simulink model "sm_abbYuMi_trajectory"  (R2025a)
settings: Solver=daessc  StartTime=0.0  StopTime=size(waypointsL,2)*segment_duration  MaxStep=0.5  RelTol=1e-3  AbsTol=1e-3
values from neighbouring files (symbols this model uses):
  cube_l = 0.02    [startup_sm_abbYuMi_trajectory.m]
  segment_duration = 2    [startup_sm_abbYuMi_trajectory.m]
undefined symbols (not defined in the file or in its folder): F1, F2, X, Y, Z
libraries: sm_lib x210, nesl_utility x31, robotcorelib x2
(part 2 of 5)

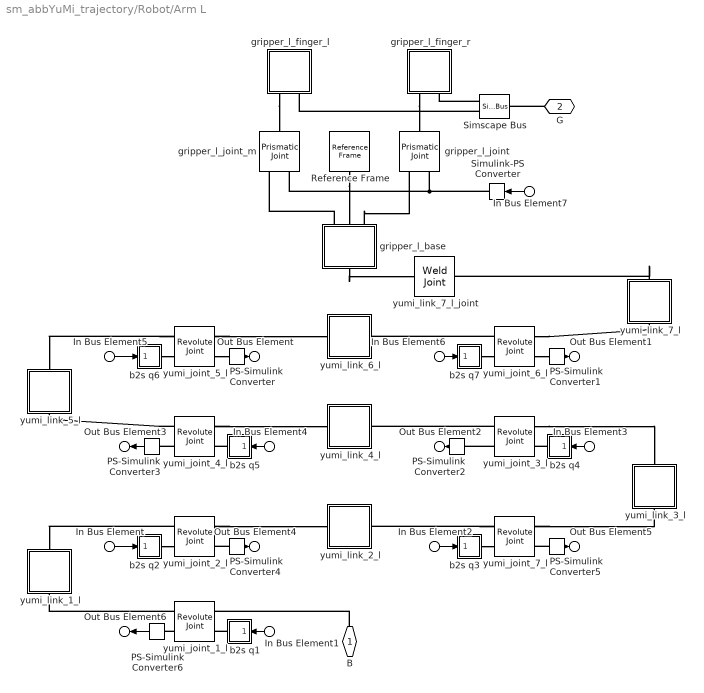
== system sm_abbYuMi_trajectory/Robot/Arm L ==
  In Bus Element1 : Inport  PortName=q  Element=q1
  In Bus Element : Inport  PortName=q  Element=q2
  In Bus Element2 : Inport  PortName=q  Element=q3
  In Bus Element3 : Inport  PortName=q  Element=q4
  In Bus Element4 : Inport  PortName=q  Element=q5
  In Bus Element5 : Inport  PortName=q  Element=q6
  In Bus Element6 : Inport  PortName=q  Element=q7
  In Bus Element7 : Inport  PortName=q  Element=f
  PS-Simulink Converter{,1..6} (7 alike) : nesl_utility/PS-Simulink Converter  PhysicalDomain=network_engine_domain  SubClassName=ps_output  LeftPortType=input  RightPortType=output  PseudoPeriodic=off  Frequencies=[]  VectorFormat=1-D array  Unit=inherit  AffineConversion=off
  Reference Frame : sm_lib/Frames and Transforms/Reference Frame
  Simscape Bus : SimscapeBus  HierarchyStrings=F1;F2
  Simulink-PS Converter : nesl_utility/Simulink-PS Converter  PhysicalDomain=network_engine_domain  SubClassName=ps_input  LeftPortType=input  RightPortType=output  PseudoPeriodic=off  Frequencies=[]  NoiseDistribution=none  NoiseParameters=[]  Unit=m  AffineConversion=off  FilteringAndDerivatives=filter  SimscapeFilterOrder=2  InputFilterTimeConstant=0.1  UdotUserProvided=0
  b2s q1 : Subsystem
  b2s q2 : Subsystem
  b2s q3 : Subsystem
  b2s q4 : Subsystem
  b2s q5 : Subsystem
  b2s q6 : Subsystem
  b2s q7 : Subsystem
  gripper_l_base : Subsystem
  gripper_l_finger_l : Subsystem
  gripper_l_finger_r : Subsystem
  gripper_l_joint : sm_lib/Joints/Prismatic Joint  JointMode=Normal  CompositeWrenchDir=FollowerOnBase  CompositeWrenchFrame=BaseFrame  SenseConstraintForce=off  SenseConstraintTorque=off  SenseTotalForce=off  SenseTotalTorque=off  PositionTargetSpecify=off  PositionTargetPriority=High  PositionTargetValue=0  PositionTargetValueUnits=m  VelocityTargetSpecify=off  VelocityTargetPriority=High  VelocityTargetValue=0  VelocityTargetValueUnits=m/s  EquilibriumPosition=0  EquilibriumPositionUnits=m  SpringStiffness=0  SpringStiffnessUnits=N/m  DampingCoefficient=1  DampingCoefficientUnits=kg/s  LowerLimitSpecify=on  LowerLimitBound=0  LowerLimitBoundUnits=m  LowerLimitStiffness=1e6  LowerLimitStiffnessUnits=N/m  LowerLimitDamping=1e3  LowerLimitDampingUnits=N/(m/s)  LowerLimitTransitionRegionWidth=1e-4  LowerLimitTransitionRegionWidthUnits=m  UpperLimitSpecify=on  UpperLimitBound=0.025  UpperLimitBoundUnits=m  UpperLimitStiffness=1e6  UpperLimitStiffnessUnits=N/m  UpperLimitDamping=1e3  UpperLimitDampingUnits=N/(m/s)  UpperLimitTransitionRegionWidth=1e-4  UpperLimitTransitionRegionWidthUnits=m  TorqueActuationMode=ComputedTorque  MotionActuationMode=InputMotion  SensePosition=off  SenseVelocity=off  SenseAcceleration=off  SenseTorqueForce=off  SenseLowerLimitTorqueForce=off  SenseUpperLimitTorqueForce=off
  gripper_l_joint_m : sm_lib/Joints/Prismatic Joint  JointMode=Normal  CompositeWrenchDir=FollowerOnBase  CompositeWrenchFrame=BaseFrame  SenseConstraintForce=off  SenseConstraintTorque=off  SenseTotalForce=off  SenseTotalTorque=off  PositionTargetSpecify=off  PositionTargetPriority=High  PositionTargetValue=0  PositionTargetValueUnits=m  VelocityTargetSpecify=off  VelocityTargetPriority=High  VelocityTargetValue=0  VelocityTargetValueUnits=m/s  EquilibriumPosition=0  EquilibriumPositionUnits=m  SpringStiffness=0  SpringStiffnessUnits=N/m  DampingCoefficient=1  DampingCoefficientUnits=kg/s  LowerLimitSpecify=on  LowerLimitBound=0  LowerLimitBoundUnits=m  LowerLimitStiffness=1e6  LowerLimitStiffnessUnits=N/m  LowerLimitDamping=1e3  LowerLimitDampingUnits=N/(m/s)  LowerLimitTransitionRegionWidth=1e-4  LowerLimitTransitionRegionWidthUnits=m  UpperLimitSpecify=on  UpperLimitBound=0.025  UpperLimitBoundUnits=m  UpperLimitStiffness=1e6  UpperLimitStiffnessUnits=N/m  UpperLimitDamping=1e3  UpperLimitDampingUnits=N/(m/s)  UpperLimitTransitionRegionWidth=1e-4  UpperLimitTransitionRegionWidthUnits=m  TorqueActuationMode=ComputedTorque  MotionActuationMode=InputMotion  SensePosition=off  SenseVelocity=off  SenseAcceleration=off  SenseTorqueForce=off  SenseLowerLimitTorqueForce=off  SenseUpperLimitTorqueForce=off
  yumi_joint_1_l : sm_lib/Joints/Revolute Joint  JointMode=Normal  CompositeWrenchDir=FollowerOnBase  CompositeWrenchFrame=BaseFrame  SenseConstraintForce=off  SenseConstraintTorque=off  SenseTotalForce=off  SenseTotalTorque=off  PositionTargetSpecify=on  PositionTargetPriority=High  PositionTargetValue=45  PositionTargetValueUnits=deg  VelocityTargetSpecify=off  VelocityTargetPriority=High  VelocityTargetValue=0  VelocityTargetValueUnits=deg/s  EquilibriumPosition=0  EquilibriumPositionUnits=deg  SpringStiffness=0  SpringStiffnessUnits=N*m/deg  DampingCoefficient=0.5  DampingCoefficientUnits=m^2*kg/s/rad  LowerLimitSpecify=on  LowerLimitBound=-2.94087978961  LowerLimitBoundUnits=rad  LowerLimitStiffness=1e4  LowerLimitStiffnessUnits=N*m/deg  LowerLimitDamping=10  LowerLimitDampingUnits=N*m/(deg/s)  LowerLimitTransitionRegionWidth=0.1  LowerLimitTransitionRegionWidthUnits=deg  UpperLimitSpecify=on  UpperLimitBound=2.94087978961  UpperLimitBoundUnits=rad  UpperLimitStiffness=1e4  UpperLimitStiffnessUnits=N*m/deg  UpperLimitDamping=10  UpperLimitDampingUnits=N*m/(deg/s)  UpperLimitTransitionRegionWidth=0.1  UpperLimitTransitionRegionWidthUnits=deg  TorqueActuationMode=ComputedTorque  MotionActuationMode=InputMotion  SensePosition=off  SenseVelocity=off  SenseAcceleration=off  SenseTorqueForce=on  SenseLowerLimitTorqueForce=off  SenseUpperLimitTorqueForce=off
  yumi_joint_2_l : sm_lib/Joints/Revolute Joint  JointMode=Normal  CompositeWrenchDir=FollowerOnBase  CompositeWrenchFrame=BaseFrame  SenseConstraintForce=off  SenseConstraintTorque=off  SenseTotalForce=off  SenseTotalTorque=off  PositionTargetSpecify=off  PositionTargetPriority=High  PositionTargetValue=0  PositionTargetValueUnits=deg  VelocityTargetSpecify=off  VelocityTargetPriority=High  VelocityTargetValue=0  VelocityTargetValueUnits=deg/s  EquilibriumPosition=0  EquilibriumPositionUnits=deg  SpringStiffness=0  SpringStiffnessUnits=N*m/deg  DampingCoefficient=0.5  DampingCoefficientUnits=m^2*kg/s/rad  LowerLimitSpecify=on  LowerLimitBound=-2.50454747661  LowerLimitBoundUnits=rad  LowerLimitStiffness=1e4  LowerLimitStiffnessUnits=N*m/deg  LowerLimitDamping=10  LowerLimitDampingUnits=N*m/(deg/s)  LowerLimitTransitionRegionWidth=0.1  LowerLimitTransitionRegionWidthUnits=deg  UpperLimitSpecify=on  UpperLimitBound=0.759218224618  UpperLimitBoundUnits=rad  UpperLimitStiffness=1e4  UpperLimitStiffnessUnits=N*m/deg  UpperLimitDamping=10  UpperLimitDampingUnits=N*m/(deg/s)  UpperLimitTransitionRegionWidth=0.1  UpperLimitTransitionRegionWidthUnits=deg  TorqueActuationMode=ComputedTorque  MotionActuationMode=InputMotion  SensePosition=off  SenseVelocity=off  SenseAcceleration=off  SenseTorqueForce=on  SenseLowerLimitTorqueForce=off  SenseUpperLimitTorqueForce=off
  yumi_joint_3_l : sm_lib/Joints/Revolute Joint  JointMode=Normal  CompositeWrenchDir=FollowerOnBase  CompositeWrenchFrame=BaseFrame  SenseConstraintForce=off  SenseConstraintTorque=off  SenseTotalForce=off  SenseTotalTorque=off  PositionTargetSpecify=off  PositionTargetPriority=High  PositionTargetValue=0  PositionTargetValueUnits=deg  VelocityTargetSpecify=off  VelocityTargetPriority=High  VelocityTargetValue=0  VelocityTargetValueUnits=deg/s  EquilibriumPosition=0  EquilibriumPositionUnits=deg  SpringStiffness=0  SpringStiffnessUnits=N*m/deg  DampingCoefficient=0.5  DampingCoefficientUnits=m^2*kg/s/rad  LowerLimitSpecify=on  LowerLimitBound=-2.15548162621  LowerLimitBoundUnits=rad  LowerLimitStiffness=1e4  LowerLimitStiffnessUnits=N*m/deg  LowerLimitDamping=10  LowerLimitDampingUnits=N*m/(deg/s)  LowerLimitTransitionRegionWidth=0.1  LowerLimitTransitionRegionWidthUnits=deg  UpperLimitSpecify=on  UpperLimitBound=1.3962634016  UpperLimitBoundUnits=rad  UpperLimitStiffness=1e4  UpperLimitStiffnessUnits=N*m/deg  UpperLimitDamping=10  UpperLimitDampingUnits=N*m/(deg/s)  UpperLimitTransitionRegionWidth=0.1  UpperLimitTransitionRegionWidthUnits=deg  TorqueActuationMode=ComputedTorque  MotionActuationMode=InputMotion  SensePosition=off  SenseVelocity=off  SenseAcceleration=off  SenseTorqueForce=on  SenseLowerLimitTorqueForce=off  SenseUpperLimitTorqueForce=off
  yumi_joint_4_l : sm_lib/Joints/Revolute Joint  JointMode=Normal  CompositeWrenchDir=FollowerOnBase  CompositeWrenchFrame=BaseFrame  SenseConstraintForce=off  SenseConstraintTorque=off  SenseTotalForce=off  SenseTotalTorque=off  PositionTargetSpecify=off  PositionTargetPriority=High  PositionTargetValue=0  PositionTargetValueUnits=deg  VelocityTargetSpecify=off  VelocityTargetPriority=High  VelocityTargetValue=0  VelocityTargetValueUnits=deg/s  EquilibriumPosition=0  EquilibriumPositionUnits=deg  SpringStiffness=0  SpringStiffnessUnits=N*m/deg  DampingCoefficient=0.5  DampingCoefficientUnits=m^2*kg/s/rad  LowerLimitSpecify=on  LowerLimitBound=-5.06145483078  LowerLimitBoundUnits=rad  LowerLimitStiffness=1e4  LowerLimitStiffnessUnits=N*m/deg  LowerLimitDamping=10  LowerLimitDampingUnits=N*m/(deg/s)  LowerLimitTransitionRegionWidth=0.1  LowerLimitTransitionRegionWidthUnits=deg  UpperLimitSpecify=on  UpperLimitBound=5.06145483078  UpperLimitBoundUnits=rad  UpperLimitStiffness=1e4  UpperLimitStiffnessUnits=N*m/deg  UpperLimitDamping=10  UpperLimitDampingUnits=N*m/(deg/s)  UpperLimitTransitionRegionWidth=0.1  UpperLimitTransitionRegionWidthUnits=deg  TorqueActuationMode=ComputedTorque  MotionActuationMode=InputMotion  SensePosition=off  SenseVelocity=off  SenseAcceleration=off  SenseTorqueForce=on  SenseLowerLimitTorqueForce=off  SenseUpperLimitTorqueForce=off
  yumi_joint_5_l : sm_lib/Joints/Revolute Joint  JointMode=Normal  CompositeWrenchDir=FollowerOnBase  CompositeWrenchFrame=BaseFrame  SenseConstraintForce=off  SenseConstraintTorque=off  SenseTotalForce=off  SenseTotalTorque=off  PositionTargetSpecify=off  PositionTargetPriority=High  PositionTargetValue=0  PositionTargetValueUnits=deg  VelocityTargetSpecify=off  VelocityTargetPriority=High  VelocityTargetValue=0  VelocityTargetValueUnits=deg/s  EquilibriumPosition=0  EquilibriumPositionUnits=deg  SpringStiffness=0  SpringStiffnessUnits=N*m/deg  DampingCoefficient=0.5  DampingCoefficientUnits=m^2*kg/s/rad  LowerLimitSpecify=on  LowerLimitBound=-1.53588974176  LowerLimitBoundUnits=rad  LowerLimitStiffness=1e4  LowerLimitStiffnessUnits=N*m/deg  LowerLimitDamping=10  LowerLimitDampingUnits=N*m/(deg/s)  LowerLimitTransitionRegionWidth=0.1  LowerLimitTransitionRegionWidthUnits=deg  UpperLimitSpecify=on  UpperLimitBound=2.40855436775  UpperLimitBoundUnits=rad  UpperLimitStiffness=1e4  UpperLimitStiffnessUnits=N*m/deg  UpperLimitDamping=10  UpperLimitDampingUnits=N*m/(deg/s)  UpperLimitTransitionRegionWidth=0.1  UpperLimitTransitionRegionWidthUnits=deg  TorqueActuationMode=ComputedTorque  MotionActuationMode=InputMotion  SensePosition=off  SenseVelocity=off  SenseAcceleration=off  SenseTorqueForce=on  SenseLowerLimitTorqueForce=off  SenseUpperLimitTorqueForce=off
  yumi_joint_6_l : sm_lib/Joints/Revolute Joint  JointMode=Normal  CompositeWrenchDir=FollowerOnBase  CompositeWrenchFrame=BaseFrame  SenseConstraintForce=off  SenseConstraintTorque=off  SenseTotalForce=off  SenseTotalTorque=off  PositionTargetSpecify=off  PositionTargetPriority=High  PositionTargetValue=0  PositionTargetValueUnits=deg  VelocityTargetSpecify=off  VelocityTargetPriority=High  VelocityTargetValue=0  VelocityTargetValueUnits=deg/s  EquilibriumPosition=0  EquilibriumPositionUnits=deg  SpringStiffness=0  SpringStiffnessUnits=N*m/deg  DampingCoefficient=0.5  DampingCoefficientUnits=m^2*kg/s/rad  LowerLimitSpecify=on  LowerLimitBound=-3.99680398707  LowerLimitBoundUnits=rad  LowerLimitStiffness=1e4  LowerLimitStiffnessUnits=N*m/deg  LowerLimitDamping=10  LowerLimitDampingUnits=N*m/(deg/s)  LowerLimitTransitionRegionWidth=0.1  LowerLimitTransitionRegionWidthUnits=deg  UpperLimitSpecify=on  UpperLimitBound=3.99680398707  UpperLimitBoundUnits=rad  UpperLimitStiffness=1e4  UpperLimitStiffnessUnits=N*m/deg  UpperLimitDamping=10  UpperLimitDampingUnits=N*m/(deg/s)  UpperLimitTransitionRegionWidth=0.1  UpperLimitTransitionRegionWidthUnits=deg  TorqueActuationMode=ComputedTorque  MotionActuationMode=InputMotion  SensePosition=off  SenseVelocity=off  SenseAcceleration=off  SenseTorqueForce=on  SenseLowerLimitTorqueForce=off  SenseUpperLimitTorqueForce=off
  yumi_joint_7_l : sm_lib/Joints/Revolute Joint  JointMode=Normal  CompositeWrenchDir=FollowerOnBase  CompositeWrenchFrame=BaseFrame  SenseConstraintForce=off  SenseConstraintTorque=off  SenseTotalForce=off  SenseTotalTorque=off  PositionTargetSpecify=off  PositionTargetPriority=High  PositionTargetValue=0  PositionTargetValueUnits=deg  VelocityTargetSpecify=off  VelocityTargetPriority=High  VelocityTargetValue=0  VelocityTargetValueUnits=deg/s  EquilibriumPosition=0  EquilibriumPositionUnits=deg  SpringStiffness=0  SpringStiffnessUnits=N*m/deg  DampingCoefficient=0.5  DampingCoefficientUnits=m^2*kg/s/rad  LowerLimitSpecify=on  LowerLimitBound=-2.94087978961  LowerLimitBoundUnits=rad  LowerLimitStiffness=1e4  LowerLimitStiffnessUnits=N*m/deg  LowerLimitDamping=10  LowerLimitDampingUnits=N*m/(deg/s)  LowerLimitTransitionRegionWidth=0.1  LowerLimitTransitionRegionWidthUnits=deg  UpperLimitSpecify=on  UpperLimitBound=2.94087978961  UpperLimitBoundUnits=rad  UpperLimitStiffness=1e4  UpperLimitStiffnessUnits=N*m/deg  UpperLimitDamping=10  UpperLimitDampingUnits=N*m/(deg/s)  UpperLimitTransitionRegionWidth=0.1  UpperLimitTransitionRegionWidthUnits=deg  TorqueActuationMode=ComputedTorque  MotionActuationMode=InputMotion  SensePosition=off  SenseVelocity=off  SenseAcceleration=off  SenseTorqueForce=on  SenseLowerLimitTorqueForce=off  SenseUpperLimitTorqueForce=off
  yumi_link_1_l : Subsystem
  yumi_link_2_l : Subsystem
  yumi_link_3_l : Subsystem
  yumi_link_4_l : Subsystem
  yumi_link_5_l : Subsystem
  yumi_link_6_l : Subsystem
  yumi_link_7_l : Subsystem
  yumi_link_7_l_joint : sm_lib/Joints/Weld Joint  JointMode=Normal  CompositeWrenchDir=FollowerOnBase  CompositeWrenchFrame=BaseFrame  SenseConstraintForce=off  SenseConstraintTorque=off  SenseTotalForce=off  SenseTotalTorque=off
  B : PMIOPort  Side=Right
  G : PMIOPort  Port=2  Side=Right
  Out Bus Element : Outport  PortName=trq  Element=j6
  Out Bus Element1 : Outport  PortName=trq  Element=j7
  Out Bus Element2 : Outport  PortName=trq  Element=j4
  Out Bus Element3 : Outport  PortName=trq  Element=j5
  Out Bus Element4 : Outport  PortName=trq  Element=j2
  Out Bus Element5 : Outport  PortName=trq  Element=j3
  Out Bus Element6 : Outport  PortName=trq  Element=j1
  wires:
  In Bus Element1/1 -> b2s q1/1(b)
  In Bus Element/1 -> b2s q2/1(b)
  In Bus Element2/1 -> b2s q3/1(b)
  In Bus Element3/1 -> b2s q4/1(b)
  In Bus Element4/1 -> b2s q5/1(b)
  In Bus Element5/1 -> b2s q6/1(b)
  In Bus Element6/1 -> b2s q7/1(b)
  In Bus Element7/1 -> Simulink-PS Converter/1
  PS-Simulink Converter/1 -> Out Bus Element/1
  PS-Simulink Converter1/1 -> Out Bus Element1/1
  PS-Simulink Converter2/1 -> Out Bus Element2/1
  PS-Simulink Converter3/1 -> Out Bus Element3/1
  PS-Simulink Converter4/1 -> Out Bus Element4/1
  PS-Simulink Converter5/1 -> Out Bus Element5/1
  PS-Simulink Converter6/1 -> Out Bus Element6/1
  connections:
  gripper_l_base/LConn1 -- yumi_link_7_l_joint/RConn1
  gripper_l_finger_l/LConn1 -- gripper_l_joint_m/RConn1
  gripper_l_base/RConn3 -- gripper_l_joint/LConn1
  yumi_joint_1_l/RConn1 -- yumi_link_1_l/LConn1
  yumi_joint_2_l/LConn1 -- yumi_link_1_l/RConn1
  yumi_joint_4_l/RConn1 -- yumi_link_5_l/LConn1
  yumi_link_7_l/RConn1 -- yumi_link_7_l_joint/LConn1
  yumi_joint_4_l/LConn1 -- yumi_link_4_l/RConn1
  yumi_joint_7_l/RConn1 -- yumi_link_3_l/LConn1
  yumi_joint_3_l/RConn1 -- yumi_link_4_l/LConn1
  yumi_joint_2_l/RConn1 -- yumi_link_2_l/LConn1
  yumi_joint_5_l/LConn1 -- yumi_link_5_l/RConn1
  yumi_joint_6_l/LConn1 -- yumi_link_6_l/RConn1
  yumi_joint_5_l/RConn1 -- yumi_link_6_l/LConn1
  gripper_l_base/RConn1 -- gripper_l_joint_m/LConn1
  yumi_joint_3_l/LConn1 -- yumi_link_3_l/RConn1
  gripper_l_finger_r/LConn1 -- gripper_l_joint/RConn1
  yumi_joint_7_l/LConn1 -- yumi_link_2_l/RConn1
  yumi_joint_6_l/RConn1 -- yumi_link_7_l/LConn1
  B/RConn1 -- yumi_joint_1_l/LConn1
  b2s q1/RConn1 -- yumi_joint_1_l/LConn2
  b2s q2/RConn1 -- yumi_joint_2_l/LConn2
  b2s q3/RConn1 -- yumi_joint_7_l/LConn2
  b2s q4/RConn1 -- yumi_joint_3_l/LConn2
  b2s q5/RConn1 -- yumi_joint_4_l/LConn2
  b2s q6/RConn1 -- yumi_joint_5_l/LConn2
  b2s q7/RConn1 -- yumi_joint_6_l/LConn2
  Simulink-PS Converter/RConn1 -- gripper_l_joint/LConn2 -- gripper_l_joint_m/LConn2
  Reference Frame/RConn1 -- gripper_l_base/RConn2
  G/RConn1 -- Simscape Bus/RConn1
  Simscape Bus/LConn1 -- gripper_l_finger_r/LConn2
  Simscape Bus/LConn2 -- gripper_l_finger_l/LConn2
  yumi_joint_5_l/RConn2 -- PS-Simulink Converter/LConn1
  yumi_joint_6_l/RConn2 -- PS-Simulink Converter1/LConn1
  yumi_joint_3_l/RConn2 -- PS-Simulink Converter2/LConn1
  yumi_joint_4_l/RConn2 -- PS-Simulink Converter3/LConn1
  PS-Simulink Converter4/LConn1 -- yumi_joint_2_l/RConn2
  PS-Simulink Converter5/LConn1 -- yumi_joint_7_l/RConn2
  yumi_joint_1_l/RConn2 -- PS-Simulink Converter6/LConn1

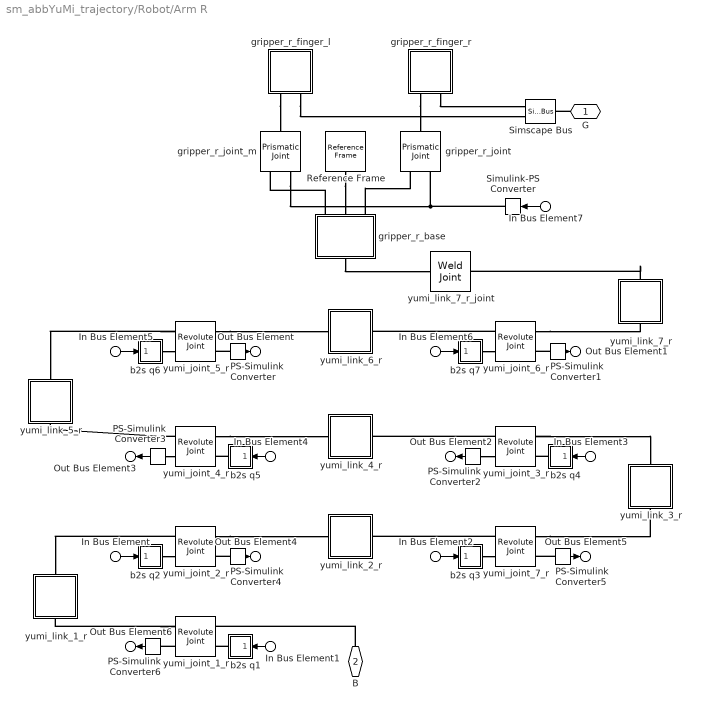
== system sm_abbYuMi_trajectory/Robot/Arm R ==
  In Bus Element1 : Inport  PortName=q  Element=q1
  In Bus Element : Inport  PortName=q  Element=q2
  In Bus Element2 : Inport  PortName=q  Element=q3
  In Bus Element3 : Inport  PortName=q  Element=q4
  In Bus Element4 : Inport  PortName=q  Element=q5
  In Bus Element5 : Inport  PortName=q  Element=q6
  In Bus Element6 : Inport  PortName=q  Element=q7
  In Bus Element7 : Inport  PortName=q  Element=f
  PS-Simulink Converter{,1..6} (7 alike) : nesl_utility/PS-Simulink Converter  PhysicalDomain=network_engine_domain  SubClassName=ps_output  LeftPortType=input  RightPortType=output  PseudoPeriodic=off  Frequencies=[]  VectorFormat=1-D array  Unit=inherit  AffineConversion=off
  Reference Frame : sm_lib/Frames and Transforms/Reference Frame
  Simscape Bus : SimscapeBus  HierarchyStrings=F1;F2
  Simulink-PS Converter : nesl_utility/Simulink-PS Converter  PhysicalDomain=network_engine_domain  SubClassName=ps_input  LeftPortType=input  RightPortType=output  PseudoPeriodic=off  Frequencies=[]  NoiseDistribution=none  NoiseParameters=[]  Unit=m  AffineConversion=off  FilteringAndDerivatives=filter  SimscapeFilterOrder=2  InputFilterTimeConstant=0.1  UdotUserProvided=0
  b2s q1 : Subsystem
  b2s q2 : Subsystem
  b2s q3 : Subsystem
  b2s q4 : Subsystem
  b2s q5 : Subsystem
  b2s q6 : Subsystem
  b2s q7 : Subsystem
  gripper_r_base : Subsystem
  gripper_r_finger_l : Subsystem
  gripper_r_finger_r : Subsystem
  gripper_r_joint : sm_lib/Joints/Prismatic Joint  JointMode=Normal  CompositeWrenchDir=FollowerOnBase  CompositeWrenchFrame=BaseFrame  SenseConstraintForce=off  SenseConstraintTorque=off  SenseTotalForce=off  SenseTotalTorque=off  PositionTargetSpecify=off  PositionTargetPriority=High  PositionTargetValue=0  PositionTargetValueUnits=m  VelocityTargetSpecify=off  VelocityTargetPriority=High  VelocityTargetValue=0  VelocityTargetValueUnits=m/s  EquilibriumPosition=0  EquilibriumPositionUnits=m  SpringStiffness=0  SpringStiffnessUnits=N/m  DampingCoefficient=1  DampingCoefficientUnits=kg/s  LowerLimitSpecify=on  LowerLimitBound=0  LowerLimitBoundUnits=m  LowerLimitStiffness=1e6  LowerLimitStiffnessUnits=N/m  LowerLimitDamping=1e3  LowerLimitDampingUnits=N/(m/s)  LowerLimitTransitionRegionWidth=1e-4  LowerLimitTransitionRegionWidthUnits=m  UpperLimitSpecify=on  UpperLimitBound=0.025  UpperLimitBoundUnits=m  UpperLimitStiffness=1e6  UpperLimitStiffnessUnits=N/m  UpperLimitDamping=1e3  UpperLimitDampingUnits=N/(m/s)  UpperLimitTransitionRegionWidth=1e-4  UpperLimitTransitionRegionWidthUnits=m  TorqueActuationMode=ComputedTorque  MotionActuationMode=InputMotion  SensePosition=off  SenseVelocity=off  SenseAcceleration=off  SenseTorqueForce=off  SenseLowerLimitTorqueForce=off  SenseUpperLimitTorqueForce=off
  gripper_r_joint_m : sm_lib/Joints/Prismatic Joint  JointMode=Normal  CompositeWrenchDir=FollowerOnBase  CompositeWrenchFrame=BaseFrame  SenseConstraintForce=off  SenseConstraintTorque=off  SenseTotalForce=off  SenseTotalTorque=off  PositionTargetSpecify=off  PositionTargetPriority=High  PositionTargetValue=0  PositionTargetValueUnits=m  VelocityTargetSpecify=off  VelocityTargetPriority=High  VelocityTargetValue=0  VelocityTargetValueUnits=m/s  EquilibriumPosition=0  EquilibriumPositionUnits=m  SpringStiffness=0  SpringStiffnessUnits=N/m  DampingCoefficient=1  DampingCoefficientUnits=kg/s  LowerLimitSpecify=on  LowerLimitBound=0  LowerLimitBoundUnits=m  LowerLimitStiffness=1e6  LowerLimitStiffnessUnits=N/m  LowerLimitDamping=1e3  LowerLimitDampingUnits=N/(m/s)  LowerLimitTransitionRegionWidth=1e-4  LowerLimitTransitionRegionWidthUnits=m  UpperLimitSpecify=on  UpperLimitBound=0.025  UpperLimitBoundUnits=m  UpperLimitStiffness=1e6  UpperLimitStiffnessUnits=N/m  UpperLimitDamping=1e3  UpperLimitDampingUnits=N/(m/s)  UpperLimitTransitionRegionWidth=1e-4  UpperLimitTransitionRegionWidthUnits=m  TorqueActuationMode=ComputedTorque  MotionActuationMode=InputMotion  SensePosition=off  SenseVelocity=off  SenseAcceleration=off  SenseTorqueForce=off  SenseLowerLimitTorqueForce=off  SenseUpperLimitTorqueForce=off
  yumi_joint_1_r : sm_lib/Joints/Revolute Joint  JointMode=Normal  CompositeWrenchDir=FollowerOnBase  CompositeWrenchFrame=BaseFrame  SenseConstraintForce=off  SenseConstraintTorque=off  SenseTotalForce=off  SenseTotalTorque=off  PositionTargetSpecify=on  PositionTargetPriority=High  PositionTargetValue=-45  PositionTargetValueUnits=deg  VelocityTargetSpecify=off  VelocityTargetPriority=High  VelocityTargetValue=0  VelocityTargetValueUnits=deg/s  EquilibriumPosition=0  EquilibriumPositionUnits=deg  SpringStiffness=0  SpringStiffnessUnits=N*m/deg  DampingCoefficient=0.5  DampingCoefficientUnits=m^2*kg/s/rad  LowerLimitSpecify=on  LowerLimitBound=-2.94087978961  LowerLimitBoundUnits=rad  LowerLimitStiffness=1e4  LowerLimitStiffnessUnits=N*m/deg  LowerLimitDamping=10  LowerLimitDampingUnits=N*m/(deg/s)  LowerLimitTransitionRegionWidth=0.1  LowerLimitTransitionRegionWidthUnits=deg  UpperLimitSpecify=on  UpperLimitBound=2.94087978961  UpperLimitBoundUnits=rad  UpperLimitStiffness=1e4  UpperLimitStiffnessUnits=N*m/deg  UpperLimitDamping=10  UpperLimitDampingUnits=N*m/(deg/s)  UpperLimitTransitionRegionWidth=0.1  UpperLimitTransitionRegionWidthUnits=deg  TorqueActuationMode=ComputedTorque  MotionActuationMode=InputMotion  SensePosition=off  SenseVelocity=off  SenseAcceleration=off  SenseTorqueForce=on  SenseLowerLimitTorqueForce=off  SenseUpperLimitTorqueForce=off
  yumi_joint_2_r : sm_lib/Joints/Revolute Joint  JointMode=Normal  CompositeWrenchDir=FollowerOnBase  CompositeWrenchFrame=BaseFrame  SenseConstraintForce=off  SenseConstraintTorque=off  SenseTotalForce=off  SenseTotalTorque=off  PositionTargetSpecify=off  PositionTargetPriority=High  PositionTargetValue=0  PositionTargetValueUnits=deg  VelocityTargetSpecify=off  VelocityTargetPriority=High  VelocityTargetValue=0  VelocityTargetValueUnits=deg/s  EquilibriumPosition=0  EquilibriumPositionUnits=deg  SpringStiffness=0  SpringStiffnessUnits=N*m/deg  DampingCoefficient=0.5  DampingCoefficientUnits=m^2*kg/s/rad  LowerLimitSpecify=on  LowerLimitBound=-2.50454747661  LowerLimitBoundUnits=rad  LowerLimitStiffness=1e4  LowerLimitStiffnessUnits=N*m/deg  LowerLimitDamping=10  LowerLimitDampingUnits=N*m/(deg/s)  LowerLimitTransitionRegionWidth=0.1  LowerLimitTransitionRegionWidthUnits=deg  UpperLimitSpecify=on  UpperLimitBound=0.759218224618  UpperLimitBoundUnits=rad  UpperLimitStiffness=1e4  UpperLimitStiffnessUnits=N*m/deg  UpperLimitDamping=10  UpperLimitDampingUnits=N*m/(deg/s)  UpperLimitTransitionRegionWidth=0.1  UpperLimitTransitionRegionWidthUnits=deg  TorqueActuationMode=ComputedTorque  MotionActuationMode=InputMotion  SensePosition=off  SenseVelocity=off  SenseAcceleration=off  SenseTorqueForce=on  SenseLowerLimitTorqueForce=off  SenseUpperLimitTorqueForce=off
  yumi_joint_3_r : sm_lib/Joints/Revolute Joint  JointMode=Normal  CompositeWrenchDir=FollowerOnBase  CompositeWrenchFrame=BaseFrame  SenseConstraintForce=off  SenseConstraintTorque=off  SenseTotalForce=off  SenseTotalTorque=off  PositionTargetSpecify=off  PositionTargetPriority=High  PositionTargetValue=0  PositionTargetValueUnits=deg  VelocityTargetSpecify=off  VelocityTargetPriority=High  VelocityTargetValue=0  VelocityTargetValueUnits=deg/s  EquilibriumPosition=0  EquilibriumPositionUnits=deg  SpringStiffness=0  SpringStiffnessUnits=N*m/deg  DampingCoefficient=0.5  DampingCoefficientUnits=m^2*kg/s/rad  LowerLimitSpecify=on  LowerLimitBound=-2.15548162621  LowerLimitBoundUnits=rad  LowerLimitStiffness=1e4  LowerLimitStiffnessUnits=N*m/deg  LowerLimitDamping=10  LowerLimitDampingUnits=N*m/(deg/s)  LowerLimitTransitionRegionWidth=0.1  LowerLimitTransitionRegionWidthUnits=deg  UpperLimitSpecify=on  UpperLimitBound=1.3962634016  UpperLimitBoundUnits=rad  UpperLimitStiffness=1e4  UpperLimitStiffnessUnits=N*m/deg  UpperLimitDamping=10  UpperLimitDampingUnits=N*m/(deg/s)  UpperLimitTransitionRegionWidth=0.1  UpperLimitTransitionRegionWidthUnits=deg  TorqueActuationMode=ComputedTorque  MotionActuationMode=InputMotion  SensePosition=off  SenseVelocity=off  SenseAcceleration=off  SenseTorqueForce=on  SenseLowerLimitTorqueForce=off  SenseUpperLimitTorqueForce=off
  yumi_joint_4_r : sm_lib/Joints/Revolute Joint  JointMode=Normal  CompositeWrenchDir=FollowerOnBase  CompositeWrenchFrame=BaseFrame  SenseConstraintForce=off  SenseConstraintTorque=off  SenseTotalForce=off  SenseTotalTorque=off  PositionTargetSpecify=off  PositionTargetPriority=High  PositionTargetValue=0  PositionTargetValueUnits=deg  VelocityTargetSpecify=off  VelocityTargetPriority=High  VelocityTargetValue=0  VelocityTargetValueUnits=deg/s  EquilibriumPosition=0  EquilibriumPositionUnits=deg  SpringStiffness=0  SpringStiffnessUnits=N*m/deg  DampingCoefficient=0.5  DampingCoefficientUnits=m^2*kg/s/rad  LowerLimitSpecify=on  LowerLimitBound=-5.06145483078  LowerLimitBoundUnits=rad  LowerLimitStiffness=1e4  LowerLimitStiffnessUnits=N*m/deg  LowerLimitDamping=10  LowerLimitDampingUnits=N*m/(deg/s)  LowerLimitTransitionRegionWidth=0.1  LowerLimitTransitionRegionWidthUnits=deg  UpperLimitSpecify=on  UpperLimitBound=5.06145483078  UpperLimitBoundUnits=rad  UpperLimitStiffness=1e4  UpperLimitStiffnessUnits=N*m/deg  UpperLimitDamping=10  UpperLimitDampingUnits=N*m/(deg/s)  UpperLimitTransitionRegionWidth=0.1  UpperLimitTransitionRegionWidthUnits=deg  TorqueActuationMode=ComputedTorque  MotionActuationMode=InputMotion  SensePosition=off  SenseVelocity=off  SenseAcceleration=off  SenseTorqueForce=on  SenseLowerLimitTorqueForce=off  SenseUpperLimitTorqueForce=off
  yumi_joint_5_r : sm_lib/Joints/Revolute Joint  JointMode=Normal  CompositeWrenchDir=FollowerOnBase  CompositeWrenchFrame=BaseFrame  SenseConstraintForce=off  SenseConstraintTorque=off  SenseTotalForce=off  SenseTotalTorque=off  PositionTargetSpecify=off  PositionTargetPriority=High  PositionTargetValue=0  PositionTargetValueUnits=deg  VelocityTargetSpecify=off  VelocityTargetPriority=High  VelocityTargetValue=0  VelocityTargetValueUnits=deg/s  EquilibriumPosition=0  EquilibriumPositionUnits=deg  SpringStiffness=0  SpringStiffnessUnits=N*m/deg  DampingCoefficient=0.5  DampingCoefficientUnits=m^2*kg/s/rad  LowerLimitSpecify=on  LowerLimitBound=-1.53588974176  LowerLimitBoundUnits=rad  LowerLimitStiffness=1e4  LowerLimitStiffnessUnits=N*m/deg  LowerLimitDamping=10  LowerLimitDampingUnits=N*m/(deg/s)  LowerLimitTransitionRegionWidth=0.1  LowerLimitTransitionRegionWidthUnits=deg  UpperLimitSpecify=on  UpperLimitBound=2.40855436775  UpperLimitBoundUnits=rad  UpperLimitStiffness=1e4  UpperLimitStiffnessUnits=N*m/deg  UpperLimitDamping=10  UpperLimitDampingUnits=N*m/(deg/s)  UpperLimitTransitionRegionWidth=0.1  UpperLimitTransitionRegionWidthUnits=deg  TorqueActuationMode=ComputedTorque  MotionActuationMode=InputMotion  SensePosition=off  SenseVelocity=off  SenseAcceleration=off  SenseTorqueForce=on  SenseLowerLimitTorqueForce=off  SenseUpperLimitTorqueForce=off
  yumi_joint_6_r : sm_lib/Joints/Revolute Joint  JointMode=Normal  CompositeWrenchDir=FollowerOnBase  CompositeWrenchFrame=BaseFrame  SenseConstraintForce=off  SenseConstraintTorque=off  SenseTotalForce=off  SenseTotalTorque=off  PositionTargetSpecify=off  PositionTargetPriority=High  PositionTargetValue=0  PositionTargetValueUnits=deg  VelocityTargetSpecify=off  VelocityTargetPriority=High  VelocityTargetValue=0  VelocityTargetValueUnits=deg/s  EquilibriumPosition=0  EquilibriumPositionUnits=deg  SpringStiffness=0  SpringStiffnessUnits=N*m/deg  DampingCoefficient=0.5  DampingCoefficientUnits=m^2*kg/s/rad  LowerLimitSpecify=on  LowerLimitBound=-3.99680398707  LowerLimitBoundUnits=rad  LowerLimitStiffness=1e4  LowerLimitStiffnessUnits=N*m/deg  LowerLimitDamping=10  LowerLimitDampingUnits=N*m/(deg/s)  LowerLimitTransitionRegionWidth=0.1  LowerLimitTransitionRegionWidthUnits=deg  UpperLimitSpecify=on  UpperLimitBound=3.99680398707  UpperLimitBoundUnits=rad  UpperLimitStiffness=1e4  UpperLimitStiffnessUnits=N*m/deg  UpperLimitDamping=10  UpperLimitDampingUnits=N*m/(deg/s)  UpperLimitTransitionRegionWidth=0.1  UpperLimitTransitionRegionWidthUnits=deg  TorqueActuationMode=ComputedTorque  MotionActuationMode=InputMotion  SensePosition=off  SenseVelocity=off  SenseAcceleration=off  SenseTorqueForce=on  SenseLowerLimitTorqueForce=off  SenseUpperLimitTorqueForce=off
  yumi_joint_7_r : sm_lib/Joints/Revolute Joint  JointMode=Normal  CompositeWrenchDir=FollowerOnBase  CompositeWrenchFrame=BaseFrame  SenseConstraintForce=off  SenseConstraintTorque=off  SenseTotalForce=off  SenseTotalTorque=off  PositionTargetSpecify=off  PositionTargetPriority=High  PositionTargetValue=0  PositionTargetValueUnits=deg  VelocityTargetSpecify=off  VelocityTargetPriority=High  VelocityTargetValue=0  VelocityTargetValueUnits=deg/s  EquilibriumPosition=0  EquilibriumPositionUnits=deg  SpringStiffness=0  SpringStiffnessUnits=N*m/deg  DampingCoefficient=0.5  DampingCoefficientUnits=m^2*kg/s/rad  LowerLimitSpecify=on  LowerLimitBound=-2.94087978961  LowerLimitBoundUnits=rad  LowerLimitStiffness=1e4  LowerLimitStiffnessUnits=N*m/deg  LowerLimitDamping=10  LowerLimitDampingUnits=N*m/(deg/s)  LowerLimitTransitionRegionWidth=0.1  LowerLimitTransitionRegionWidthUnits=deg  UpperLimitSpecify=on  UpperLimitBound=2.94087978961  UpperLimitBoundUnits=rad  UpperLimitStiffness=1e4  UpperLimitStiffnessUnits=N*m/deg  UpperLimitDamping=10  UpperLimitDampingUnits=N*m/(deg/s)  UpperLimitTransitionRegionWidth=0.1  UpperLimitTransitionRegionWidthUnits=deg  TorqueActuationMode=ComputedTorque  MotionActuationMode=InputMotion  SensePosition=off  SenseVelocity=off  SenseAcceleration=off  SenseTorqueForce=on  SenseLowerLimitTorqueForce=off  SenseUpperLimitTorqueForce=off
  yumi_link_1_r : Subsystem
  yumi_link_2_r : Subsystem
  yumi_link_3_r : Subsystem
  yumi_link_4_r : Subsystem
  yumi_link_5_r : Subsystem
  yumi_link_6_r : Subsystem
  yumi_link_7_r : Subsystem
  yumi_link_7_r_joint : sm_lib/Joints/Weld Joint  JointMode=Normal  CompositeWrenchDir=FollowerOnBase  CompositeWrenchFrame=BaseFrame  SenseConstraintForce=off  SenseConstraintTorque=off  SenseTotalForce=off  SenseTotalTorque=off
  G : PMIOPort  Side=Right
  B : PMIOPort  Port=2  Side=Right
  Out Bus Element : Outport  PortName=trq  Element=j6
  Out Bus Element1 : Outport  PortName=trq  Element=j7
  Out Bus Element2 : Outport  PortName=trq  Element=j4
  Out Bus Element3 : Outport  PortName=trq  Element=j5
  Out Bus Element4 : Outport  PortName=trq  Element=j2
  Out Bus Element5 : Outport  PortName=trq  Element=j3
  Out Bus Element6 : Outport  PortName=trq  Element=j1
  wires:
  In Bus Element2/1 -> b2s q3/1(b)
  In Bus Element1/1 -> b2s q1/1(b)
  In Bus Element/1 -> b2s q2/1(b)
  In Bus Element4/1 -> b2s q5/1(b)
  In Bus Element5/1 -> b2s q6/1(b)
  In Bus Element3/1 -> b2s q4/1(b)
  In Bus Element6/1 -> b2s q7/1(b)
  In Bus Element7/1 -> Simulink-PS Converter/1
  PS-Simulink Converter3/1 -> Out Bus Element3/1
  PS-Simulink Converter2/1 -> Out Bus Element2/1
  PS-Simulink Converter6/1 -> Out Bus Element6/1
  PS-Simulink Converter/1 -> Out Bus Element/1
  PS-Simulink Converter1/1 -> Out Bus Element1/1
  PS-Simulink Converter4/1 -> Out Bus Element4/1
  PS-Simulink Converter5/1 -> Out Bus Element5/1
  connections:
  yumi_joint_1_r/RConn1 -- yumi_link_1_r/LConn1
  gripper_r_finger_l/LConn1 -- gripper_r_joint_m/RConn1
  yumi_joint_2_r/RConn1 -- yumi_link_2_r/LConn1
  yumi_joint_6_r/RConn1 -- yumi_link_7_r/LConn1
  yumi_joint_2_r/LConn1 -- yumi_link_1_r/RConn1
  yumi_joint_5_r/LConn1 -- yumi_link_5_r/RConn1
  yumi_joint_4_r/RConn1 -- yumi_link_5_r/LConn1
  yumi_joint_3_r/LConn1 -- yumi_link_3_r/RConn1
  yumi_joint_3_r/RConn1 -- yumi_link_4_r/LConn1
  yumi_joint_5_r/RConn1 -- yumi_link_6_r/LConn1
  yumi_joint_7_r/RConn1 -- yumi_link_3_r/LConn1
  yumi_joint_7_r/LConn1 -- yumi_link_2_r/RConn1
  yumi_joint_4_r/LConn1 -- yumi_link_4_r/RConn1
  yumi_joint_6_r/LConn1 -- yumi_link_6_r/RConn1
  gripper_r_base/LConn1 -- yumi_link_7_r_joint/RConn1
  yumi_link_7_r/RConn1 -- yumi_link_7_r_joint/LConn1
  gripper_r_base/RConn1 -- gripper_r_joint_m/LConn1
  gripper_r_base/RConn3 -- gripper_r_joint/LConn1
  gripper_r_finger_r/LConn1 -- gripper_r_joint/RConn1
  B/RConn1 -- yumi_joint_1_r/LConn1
  b2s q4/RConn1 -- yumi_joint_3_r/LConn2
  b2s q2/RConn1 -- yumi_joint_2_r/LConn2
  b2s q7/RConn1 -- yumi_joint_6_r/LConn2
  b2s q3/RConn1 -- yumi_joint_7_r/LConn2
  b2s q6/RConn1 -- yumi_joint_5_r/LConn2
  b2s q1/RConn1 -- yumi_joint_1_r/LConn2
  Simulink-PS Converter/RConn1 -- gripper_r_joint/LConn2 -- gripper_r_joint_m/LConn2
  Reference Frame/RConn1 -- gripper_r_base/RConn2
  b2s q5/RConn1 -- yumi_joint_4_r/LConn2
  G/RConn1 -- Simscape Bus/RConn1
  gripper_r_finger_r/LConn2 -- Simscape Bus/LConn1
  gripper_r_finger_l/LConn2 -- Simscape Bus/LConn2
  yumi_joint_1_r/RConn2 -- PS-Simulink Converter6/LConn1
  PS-Simulink Converter4/LConn1 -- yumi_joint_2_r/RConn2
  PS-Simulink Converter5/LConn1 -- yumi_joint_7_r/RConn2
  PS-Simulink Converter2/LConn1 -- yumi_joint_3_r/RConn2
  PS-Simulink Converter3/LConn1 -- yumi_joint_4_r/RConn2
  PS-Simulink Converter/LConn1 -- yumi_joint_5_r/RConn2
  PS-Simulink Converter1/LConn1 -- yumi_joint_6_r/RConn2

== system sm_abbYuMi_trajectory/Robot/Block 1 ==
  Brick Solid : sm_lib/Body Elements/Brick Solid  BrickDimensions=[1 1 1]*cube_l  BrickDimensionsUnits=m  ExportEntireGeometry=on  InertiaType=CalculateFromGeometry  BasedOnType=Density  Density=1000  DensityUnits=kg/m^3  Mass=1  MassUnits=kg  CenterOfMass=[0 0 0]  CenterOfMassUnits=m  MomentsOfInertia=[1 1 1]  MomentsOfInertiaUnits=kg*m^2  ProductsOfInertia=[0 0 0]  ProductsOfInertiaUnits=kg*m^2  GraphicType=FromGeometry  MarkerShape=Sphere  MarkerSize=10  GraphicVisPropType=SimpleVisualProperties  GraphicDiffuseColor=[1.0 0.6 0.0]  GraphicOpacity=1.0  GraphicSpecularColor=[0.5 0.5 0.5 1.0]  GraphicAmbientColor=[0.15 0.15 0.15 1.0]  GraphicEmissiveColor=[0.0 0.0 0.0 1.0]  GraphicShininess=75  DoExposeReferenceFrame=on  SerializedFrames=<Frames/>
  Point Cloud : sm_lib/Curves and Surfaces/Point Cloud  CoordinatesMatrix=brick_point_cloud  CoordinatesMatrixUnits=m  GraphicType=MarkerCloud  GraphicSphereRadius=1e-3  GraphicSphereRadiusUnits=m  GraphicVisPropType=SimpleVisualProperties  GraphicDiffuseColor=[1 0 0]  GraphicOpacity=1.0  GraphicSpecularColor=[0.5 0.5 0.5 1.0]  GraphicAmbientColor=[0.15 0.15 0.15 1.0]  GraphicEmissiveColor=[0.0 0.0 0.0 1.0]  GraphicShininess=75
  G : PMIOPort  Side=Left
  R : PMIOPort  Port=2  Side=Right
  C : PMIOPort  Port=3  Side=Left
  connections:
  C/RConn1 -- Point Cloud/RConn1
  Point Cloud/LConn1 -- Brick Solid/RConn1 -- R/RConn1
  G/RConn1 -- Brick Solid/LConn1

== system sm_abbYuMi_trajectory/Robot/Block 2 ==
  Brick Solid : sm_lib/Body Elements/Brick Solid  BrickDimensions=[1 1 1]*cube_l  BrickDimensionsUnits=m  ExportEntireGeometry=on  InertiaType=CalculateFromGeometry  BasedOnType=Density  Density=1000  DensityUnits=kg/m^3  Mass=1  MassUnits=kg  CenterOfMass=[0 0 0]  CenterOfMassUnits=m  MomentsOfInertia=[1 1 1]  MomentsOfInertiaUnits=kg*m^2  ProductsOfInertia=[0 0 0]  ProductsOfInertiaUnits=kg*m^2  GraphicType=FromGeometry  MarkerShape=Sphere  MarkerSize=10  GraphicVisPropType=SimpleVisualProperties  GraphicDiffuseColor=[0.0 0.8 0.4]  GraphicOpacity=1.0  GraphicSpecularColor=[0.5 0.5 0.5 1.0]  GraphicAmbientColor=[0.15 0.15 0.15 1.0]  GraphicEmissiveColor=[0.0 0.0 0.0 1.0]  GraphicShininess=75  DoExposeReferenceFrame=on  SerializedFrames=<Frames/>
  Point Cloud : sm_lib/Curves and Surfaces/Point Cloud  CoordinatesMatrix=brick_point_cloud  CoordinatesMatrixUnits=m  GraphicType=MarkerCloud  GraphicSphereRadius=1e-3  GraphicSphereRadiusUnits=m  GraphicVisPropType=SimpleVisualProperties  GraphicDiffuseColor=[1 0 0]  GraphicOpacity=1.0  GraphicSpecularColor=[0.5 0.5 0.5 1.0]  GraphicAmbientColor=[0.15 0.15 0.15 1.0]  GraphicEmissiveColor=[0.0 0.0 0.0 1.0]  GraphicShininess=75
  R : PMIOPort  Side=Right
  G : PMIOPort  Port=2  Side=Left
  C : PMIOPort  Port=3  Side=Left
  connections:
  G/RConn1 -- Brick Solid/LConn1
  R/RConn1 -- Brick Solid/RConn1 -- Point Cloud/LConn1
  C/RConn1 -- Point Cloud/RConn1

== system sm_abbYuMi_trajectory/Robot/Body ==
  yumi_base_link : Subsystem
  yumi_base_link_to_body : sm_lib/Joints/Weld Joint  JointMode=Normal  CompositeWrenchDir=FollowerOnBase  CompositeWrenchFrame=BaseFrame  SenseConstraintForce=off  SenseConstraintTorque=off  SenseTotalForce=off  SenseTotalTorque=off
  yumi_body : Subsystem
  F1 : PMIOPort  Side=Right
  F2 : PMIOPort  Port=2  Side=Right
  F : PMIOPort  Port=3  Side=Left
  connections:
  yumi_base_link/RConn1 -- yumi_base_link_to_body/LConn1
  yumi_base_link_to_body/RConn1 -- yumi_body/LConn1
  yumi_base_link/LConn1 -- F/RConn1
  yumi_body/RConn1 -- F1/RConn1
  yumi_body/RConn2 -- F2/RConn1

== system sm_abbYuMi_trajectory/Robot/Floor ==
  Brick Solid : sm_lib/Body Elements/Brick Solid  BrickDimensions=[1 1 0.01]  BrickDimensionsUnits=m  ExportEntireGeometry=off  InertiaType=CalculateFromGeometry  BasedOnType=Density  Density=1000  DensityUnits=kg/m^3  Mass=1  MassUnits=kg  CenterOfMass=[0 0 0]  CenterOfMassUnits=m  MomentsOfInertia=[1 1 1]  MomentsOfInertiaUnits=kg*m^2  ProductsOfInertia=[0 0 0]  ProductsOfInertiaUnits=kg*m^2  GraphicType=FromGeometry  MarkerShape=Sphere  MarkerSize=10  GraphicVisPropType=SimpleVisualProperties  GraphicDiffuseColor=[0.5 0.5 0.5]  GraphicOpacity=1.0  GraphicSpecularColor=[0.5 0.5 0.5 1.0]  GraphicAmbientColor=[0.15 0.15 0.15 1.0]  GraphicEmissiveColor=[0.0 0.0 0.0 1.0]  GraphicShininess=75  DoExposeReferenceFrame=on  SerializedFrames=<Frames/>
  Rigid Transform : sm_lib/Frames and Transforms/Rigid Transform  RotationMethod=None  FollAlignAxisA=+X  BaseAlignAxisA=+Y  FollAlignAxisB=+Y  BaseAlignAxisB=+Z  RotationStandardAxis=+Z  RotationAngle=0.0  RotationAngleUnits=deg  RotationArbitraryAxis=[0 0 1]  RotationSequenceAxes=FollowerAxes  RotationSequence=XYX  RotationSequenceAngles=[0 0 0]  RotationSequenceAnglesUnits=deg  RotationMatrix=[1 0 0; 0 1 0; 0 0 1]  Quaternion=[1 0 0 0]  TranslationMethod=StandardAxis  TranslationCartesianOffset=[0 0 0]  TranslationCartesianOffsetUnits=m  TranslationStandardAxis=+Z  TranslationStandardOffset=-0.005  TranslationStandardOffsetUnits=m  TranslationROffset=0  TranslationROffsetUnits=m  TranslationThetaOffset=0  TranslationThetaOffsetUnits=deg  TranslationZOffset=0  TranslationZOffsetUnits=m
  T : PMIOPort  Side=Left
  connections:
  Brick Solid/RConn1 -- Rigid Transform/RConn1
  Rigid Transform/LConn1 -- T/RConn1

== system sm_abbYuMi_trajectory/Robot/Arm L/b2s q1 ==
  b : Inport
  Demux : Demux  Outputs=3
  Simulink-PS Converter : nesl_utility/Simulink-PS Converter  PhysicalDomain=network_engine_domain  SubClassName=ps_input  LeftPortType=input  RightPortType=output  PseudoPeriodic=off  Frequencies=[]  NoiseDistribution=none  NoiseParameters=[]  Unit=rad  AffineConversion=off  FilteringAndDerivatives=provide  SimscapeFilterOrder=1  InputFilterTimeConstant=0.001  UdotUserProvided=2
  s : PMIOPort  Side=Right
  wires:
  Demux/2 -> Simulink-PS Converter/2
  b/1 -> Demux/1
  Demux/3 -> Simulink-PS Converter/3
  Demux/1 -> Simulink-PS Converter/1
  connections:
  Simulink-PS Converter/RConn1 -- s/RConn1

== system sm_abbYuMi_trajectory/Robot/Arm L/b2s q2 ==
  b : Inport
  Demux : Demux  Outputs=3
  Simulink-PS Converter : nesl_utility/Simulink-PS Converter  PhysicalDomain=network_engine_domain  SubClassName=ps_input  LeftPortType=input  RightPortType=output  PseudoPeriodic=off  Frequencies=[]  NoiseDistribution=none  NoiseParameters=[]  Unit=rad  AffineConversion=off  FilteringAndDerivatives=provide  SimscapeFilterOrder=1  InputFilterTimeConstant=0.001  UdotUserProvided=2
  s : PMIOPort  Side=Right
  wires:
  Demux/1 -> Simulink-PS Converter/1
  Demux/3 -> Simulink-PS Converter/3
  b/1 -> Demux/1
  Demux/2 -> Simulink-PS Converter/2
  connections:
  Simulink-PS Converter/RConn1 -- s/RConn1

== system sm_abbYuMi_trajectory/Robot/Arm L/b2s q3 ==
  b : Inport
  Demux : Demux  Outputs=3
  Simulink-PS Converter : nesl_utility/Simulink-PS Converter  PhysicalDomain=network_engine_domain  SubClassName=ps_input  LeftPortType=input  RightPortType=output  PseudoPeriodic=off  Frequencies=[]  NoiseDistribution=none  NoiseParameters=[]  Unit=rad  AffineConversion=off  FilteringAndDerivatives=provide  SimscapeFilterOrder=1  InputFilterTimeConstant=0.001  UdotUserProvided=2
  s : PMIOPort  Side=Right
  wires:
  Demux/1 -> Simulink-PS Converter/1
  Demux/3 -> Simulink-PS Converter/3
  b/1 -> Demux/1
  Demux/2 -> Simulink-PS Converter/2
  connections:
  Simulink-PS Converter/RConn1 -- s/RConn1

== system sm_abbYuMi_trajectory/Robot/Arm L/b2s q4 ==
  b : Inport
  Demux : Demux  Outputs=3
  Simulink-PS Converter : nesl_utility/Simulink-PS Converter  PhysicalDomain=network_engine_domain  SubClassName=ps_input  LeftPortType=input  RightPortType=output  PseudoPeriodic=off  Frequencies=[]  NoiseDistribution=none  NoiseParameters=[]  Unit=rad  AffineConversion=off  FilteringAndDerivatives=provide  SimscapeFilterOrder=1  InputFilterTimeConstant=0.001  UdotUserProvided=2
  s : PMIOPort  Side=Right
  wires:
  Demux/2 -> Simulink-PS Converter/2
  b/1 -> Demux/1
  Demux/3 -> Simulink-PS Converter/3
  Demux/1 -> Simulink-PS Converter/1
  connections:
  Simulink-PS Converter/RConn1 -- s/RConn1

== system sm_abbYuMi_trajectory/Robot/Arm L/b2s q5 ==
  b : Inport
  Demux : Demux  Outputs=3
  Simulink-PS Converter : nesl_utility/Simulink-PS Converter  PhysicalDomain=network_engine_domain  SubClassName=ps_input  LeftPortType=input  RightPortType=output  PseudoPeriodic=off  Frequencies=[]  NoiseDistribution=none  NoiseParameters=[]  Unit=rad  AffineConversion=off  FilteringAndDerivatives=provide  SimscapeFilterOrder=1  InputFilterTimeConstant=0.001  UdotUserProvided=2
  s : PMIOPort  Side=Right
  wires:
  Demux/1 -> Simulink-PS Converter/1
  Demux/3 -> Simulink-PS Converter/3
  b/1 -> Demux/1
  Demux/2 -> Simulink-PS Converter/2
  connections:
  Simulink-PS Converter/RConn1 -- s/RConn1

== system sm_abbYuMi_trajectory/Robot/Arm L/b2s q6 ==
  b : Inport
  Demux : Demux  Outputs=3
  Simulink-PS Converter : nesl_utility/Simulink-PS Converter  PhysicalDomain=network_engine_domain  SubClassName=ps_input  LeftPortType=input  RightPortType=output  PseudoPeriodic=off  Frequencies=[]  NoiseDistribution=none  NoiseParameters=[]  Unit=rad  AffineConversion=off  FilteringAndDerivatives=provide  SimscapeFilterOrder=1  InputFilterTimeConstant=0.001  UdotUserProvided=2
  s : PMIOPort  Side=Right
  wires:
  Demux/2 -> Simulink-PS Converter/2
  b/1 -> Demux/1
  Demux/3 -> Simulink-PS Converter/3
  Demux/1 -> Simulink-PS Converter/1
  connections:
  Simulink-PS Converter/RConn1 -- s/RConn1

== system sm_abbYuMi_trajectory/Robot/Arm L/b2s q7 ==
  b : Inport
  Demux : Demux  Outputs=3
  Simulink-PS Converter : nesl_utility/Simulink-PS Converter  PhysicalDomain=network_engine_domain  SubClassName=ps_input  LeftPortType=input  RightPortType=output  PseudoPeriodic=off  Frequencies=[]  NoiseDistribution=none  NoiseParameters=[]  Unit=rad  AffineConversion=off  FilteringAndDerivatives=provide  SimscapeFilterOrder=1  InputFilterTimeConstant=0.001  UdotUserProvided=2
  s : PMIOPort  Side=Right
  wires:
  Demux/1 -> Simulink-PS Converter/1
  Demux/3 -> Simulink-PS Converter/3
  b/1 -> Demux/1
  Demux/2 -> Simulink-PS Converter/2
  connections:
  Simulink-PS Converter/RConn1 -- s/RConn1
